simulink model "FullWave"  (R2024b)
settings: Solver=VariableStepAuto  StartTime=0.0  StopTime=s*(1/f)  RelTol=1e-9
model workspace (MAT data in the model file):
  E = 72
  L = 0.5
  R = 25
  Vll_rms = 480
  alpha = 30
  f = 60
  s = 1
libraries: spsMeanLib x18, eeRmsMeasurement x18, spsCurrentMeasurementLib x9, spsDiodeLib x9, spsThyristorLib x9, spsVoltageMeasurementLib x9, simulink x3, spsSeriesRLCBranchLib x3, spsThreePhaseSourceLib x3, sps_lib x1
settings Model: Creator=Mohammed Abdelrahman  LastModifiedBy=Mohammed Abdelrahman

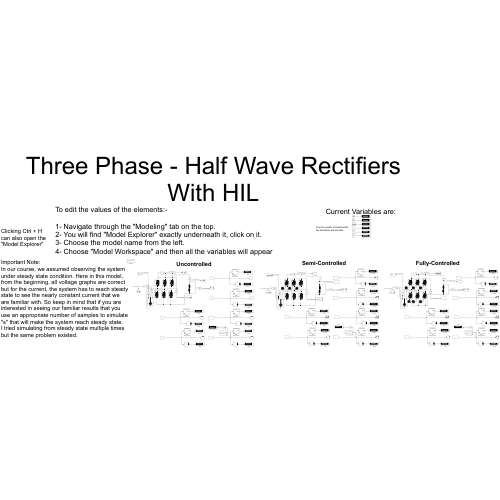
[thumbnail: Simulink's stored preview of the top-level diagram]
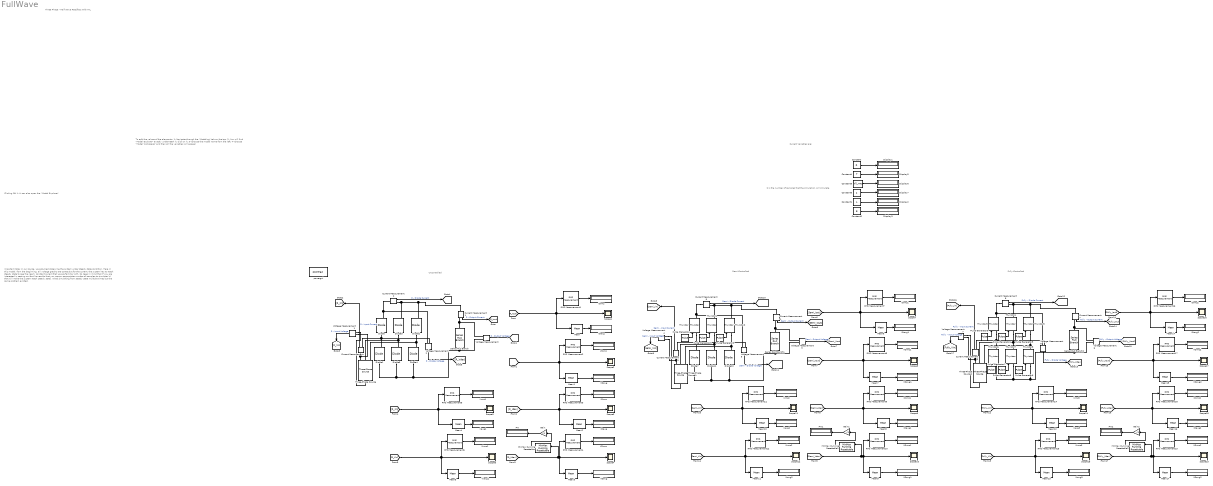
== system FullWave ==
  note: Important Note:
      | In our course, we assumed observing the system under steady state condition. Here in this model, from the beginning, all voltage graphs are correct but for the current, the system has to reach steady state to see the nearly constant current that we are familiar with. So keep in mind that if you are interested in seeing our familiar results that you use an appropriate number of samples to simulate "s" that will make the system reach steady state.
      | I tried simulating from steady state multiple times but the same problem existed.
  note: Clicking Ctrl + H can also open the "Model Explorer"
  note: S is the number of samples that the simulation will simulate
  note: Three Phase - Half Wave Rectifiers
      | With HIL
  note: To edit the values of the elements:-
      |
      | 1- Navigate through the "Modeling" tab on the top.
      | 2- You will find "Model Explorer" exactly underneath it, click on it.
      | 3- Choose the model name from the left.
      | 4- Choose "Model Workspace" and then all the variables will appear
  note: Uncontrolled
  note: Semi-Controlled
  note: Current Variables are:
  note: Fully-Controlled
  Constant : Constant  Value=R
  Constant1 : Constant  Value=L
  Constant2 : Constant  Value=E
  Constant4 : Constant  Value=f
  Constant5 : Constant  Value=Vll_rms
  Constant6 : Constant  Value=s
  Current Measurement{,1..8} (9 alike) : spsCurrentMeasurementLib/Current Measurement  PhasorSimulation=off  OutputType=Complex  PSBequivalent=0
  Diode{,1..5,7,10..11} (9 alike) : spsDiodeLib/Diode  Ron=0.001  Lon=0  Vf=0.0001  IC=0  UseSnubber=0  Rs=10e5  Cs=250e-9  Measurements=on
  Display{1..3,5..7} (6 alike) : Display
  Gain : Gain  Gain=-1
  Gain1 : Gain  Gain=-1
  Gain2 : Gain  Gain=-1
  IDavg : Display
  IDavg1 : Display
  IDavg2 : Display
  IDrms : Display
  IDrms1 : Display
  IDrms2 : Display
  IOavg : Display
  IOavg1 : Display
  IOavg2 : Display
  IOrms : Display
  IOrms1 : Display
  IOrms2 : Display
  Iiavg1 : Display
  Iiavg2 : Display
  Iiavg3 : Display
  Iirms1 : Display
  Iirms2 : Display
  Iirms3 : Display
  Mean{,1..17} (18 alike) : spsMeanLib/Mean  Freq=60  Vinit=0  Ts=0
  MinMax Running Resettable : simulink/Math Operations/MinMax Running Resettable  Function=min  vinit=0.0
  MinMax Running Resettable1 : simulink/Math Operations/MinMax Running Resettable  Function=min  vinit=0.0
  MinMax Running Resettable2 : simulink/Math Operations/MinMax Running Resettable  Function=min  vinit=0.0
  PIV : Display
  PIV1 : Display
  PIV2 : Display
  Pulse Generator : DiscretePulseGenerator  PulseType=Time based  Period=1/f  PulseWidth=5  PhaseDelay=(30+alpha)/(360*f)
  Pulse Generator1 : DiscretePulseGenerator  PulseType=Time based  Period=1/f  PulseWidth=5  PhaseDelay=(150+alpha)/(360*f)
  Pulse Generator2 : DiscretePulseGenerator  PulseType=Time based  Period=1/f  PulseWidth=5  PhaseDelay=(270+alpha)/(360*f)
  Pulse Generator3 : DiscretePulseGenerator  PulseType=Time based  Period=1/f  PulseWidth=5  PhaseDelay=(30+alpha)/(360*f)
  Pulse Generator4 : DiscretePulseGenerator  PulseType=Time based  Period=1/f  PulseWidth=5  PhaseDelay=(150+alpha)/(360*f)
  Pulse Generator5 : DiscretePulseGenerator  PulseType=Time based  Period=1/f  PulseWidth=5  PhaseDelay=(270+alpha)/(360*f)
  Pulse Generator6 : DiscretePulseGenerator  PulseType=Time based  Period=1/f  PulseWidth=5  PhaseDelay=(90+alpha)/(360*f)
  Pulse Generator7 : DiscretePulseGenerator  PulseType=Time based  Period=1/f  PulseWidth=5  PhaseDelay=(210+alpha)/(360*f)
  Pulse Generator8 : DiscretePulseGenerator  PulseType=Time based  Period=1/f  PulseWidth=5  PhaseDelay=(330+alpha)/(360*f)
  RMS Measurement{1..18} (18 alike) : eeRmsMeasurement/RMS Measurement  LabelModeActiveChoice=Total  F=f  SpecifyHarmonics=off  K=[0 1 2]  Ts=0
      settings: LibrarySourceBlock=|
      | ee_sl_lib/Measurements/RMS
      | Measurement
  Scope{1..18} (18 alike) : Scope
  Series RLC Branch : spsSeriesRLCBranchLib/Series RLC Branch  LConnTagsString=__new0  RConnTagsString=__new0  BranchType=RL  Resistance=R  Inductance=L  SetiL0=off  InitialCurrent=0  Capacitance=1e-6  Setx0=off  InitialVoltage=0  Measurements=None
  Series RLC Branch1 : spsSeriesRLCBranchLib/Series RLC Branch  LConnTagsString=__new0  RConnTagsString=__new0  BranchType=RL  Resistance=R  Inductance=L  SetiL0=off  InitialCurrent=0  Capacitance=1e-6  Setx0=off  InitialVoltage=0  Measurements=None
  Series RLC Branch2 : spsSeriesRLCBranchLib/Series RLC Branch  LConnTagsString=__new0  RConnTagsString=__new0  BranchType=RL  Resistance=R  Inductance=L  SetiL0=off  InitialCurrent=0  Capacitance=1e-6  Setx0=off  InitialVoltage=0  Measurements=None
  Three-Phase Source : spsThreePhaseSourceLib/Three-Phase Source  InternalConnection=Yn  VoltagePhases=off  Voltage=Vll_rms/sqrt(3)  PhaseAngle=0  Voltage_phases=[25e3 25e3 25e3]/sqrt(3)  PhaseAngles_phases=[0 -120 +120]  Frequency=f  NonIdealSource=off  SpecifyImpedance=off  Resistance=0.00001  Inductance=16.58e-6  ShortCircuitLevel=100e6  BaseVoltage=25e3  XRratio=7  BusType=swing  Pref=10e3  Qref=0  Prefabc=[10e3, 10e3, 10e3]  Qrefabc=[0, 0, 0]  Qmin=-inf  Qmax=inf
  Three-Phase Source1 : spsThreePhaseSourceLib/Three-Phase Source  InternalConnection=Yn  VoltagePhases=off  Voltage=Vll_rms/sqrt(3)  PhaseAngle=0  Voltage_phases=[25e3 25e3 25e3]/sqrt(3)  PhaseAngles_phases=[0 -120 +120]  Frequency=f  NonIdealSource=off  SpecifyImpedance=off  Resistance=0.00001  Inductance=16.58e-6  ShortCircuitLevel=100e6  BaseVoltage=25e3  XRratio=7  BusType=swing  Pref=10e3  Qref=0  Prefabc=[10e3, 10e3, 10e3]  Qrefabc=[0, 0, 0]  Qmin=-inf  Qmax=inf
  Three-Phase Source2 : spsThreePhaseSourceLib/Three-Phase Source  InternalConnection=Yn  VoltagePhases=off  Voltage=Vll_rms/sqrt(3)  PhaseAngle=0  Voltage_phases=[25e3 25e3 25e3]/sqrt(3)  PhaseAngles_phases=[0 -120 +120]  Frequency=f  NonIdealSource=off  SpecifyImpedance=off  Resistance=0.00001  Inductance=16.58e-6  ShortCircuitLevel=100e6  BaseVoltage=25e3  XRratio=7  BusType=swing  Pref=10e3  Qref=0  Prefabc=[10e3, 10e3, 10e3]  Qrefabc=[0, 0, 0]  Qmin=-inf  Qmax=inf
  Thyristor{,1..8} (9 alike) : spsThyristorLib/Thyristor  Ron=0.001  Lon=0  Vf=0.0001  IC=0  Rs=10e5  Cs=250e-9  Measurements=on
  VDavg : Display
  VDavg1 : Display
  VDavg2 : Display
  VDrms : Display
  VDrms1 : Display
  VDrms2 : Display
  VOavg : Display
  VOavg1 : Display
  VOavg2 : Display
  VOrms : Display
  VOrms1 : Display
  VOrms2 : Display
  Viavg1 : Display
  Viavg2 : Display
  Viavg3 : Display
  Virms1 : Display
  Virms2 : Display
  Virms3 : Display
  Voltage Measurement{,1..8} (9 alike) : spsVoltageMeasurementLib/Voltage Measurement  PhasorSimulation=off  OutputType=Complex  PSBequivalent=0
  powergui : sps_lib/powergui  Priority=1  SimulationMode=Continuous  SampleTime=50e-6  frequency=60  Iterations=50  frequencyindice=60  Pbase=100e6  ErrMax=1e-4  UnitsV=kV  UnitsW=MW  buscounter=0  FunctionMessages=off  echomessages=off  EnableUseOfTLC=off  CurrentSourceSwitches=off  DisableSnubberDevices=off  DisableRonSwitches=off  DisableVfSwitches=off  DisplayEquations=off  AutomaticDiscreteSolvers=off  SolverType=Tustin/Backward Euler (TBE)  Interpol=off  ExternalGateDelay=off  methode=off  Ts=100  x0status=steady  SPID=on  SwTol=0  HookPort=off  NonlinearTolerance=1e-4  nMaxIteration=100  ContinueOnMaxIteration=off  RestoreLinks=warning  ResistiveCurrentMeasurement=off  Frange=[0:2:500]  Ylog=off  Xlog=on  ShowGrid=off  save=off  variable=ZData  structure=0  ZoomFFT=off  StartTime=0.0  cycles=1  DisplayStyle=1  fundamental=60  FreqAxis=off  MaxFrequency=1000  frequencyindicesteady=1  RmsSteady=1  display=off
  wires:
  Current Measurement1/1 -> [R_Iout]  "R - Output Current"
  Voltage Measurement/1 -> [R_Vout]  "R - Output Voltage"
  Current Measurement/1 -> [R_Iin]  "R - Input Current"
  Voltage Measurement1/1 -> [R_Vin]  "R - Input Voltage"
  [R_Iout] -> Scope1/1, RMS Measurement1/1, Mean/1
  Mean1/1 -> VOavg/1
  Mean/1 -> IOavg/1
  [R_Vout] -> Mean1/1, RMS Measurement2/1, Scope2/1
  RMS Measurement2/1 -> VOrms/1
  RMS Measurement1/1 -> IOrms/1
  Voltage Measurement2/1 -> [R_Vdev]  "R - Diode Voltage"
  Current Measurement2/1 -> [R_Idev]  "R - Diode Current"
  [R_Vdev] -> RMS Measurement4/1, Scope4/1, Mean3/1, MinMax Running Resettable/1
  [R_Idev] -> Scope3/1, RMS Measurement3/1, Mean2/1
  RMS Measurement3/1 -> IDrms/1
  Mean3/1 -> VDavg/1
  Mean2/1 -> IDavg/1
  RMS Measurement4/1 -> VDrms/1
  Gain/1 -> PIV/1
  MinMax Running Resettable/1 -> Gain/1
  [R_Vin] -> Scope6/1, Mean5/1, RMS Measurement6/1
  [R_Iin] -> Scope5/1, RMS Measurement5/1, Mean4/1
  RMS Measurement5/1 -> Iirms1/1
  Mean5/1 -> Viavg1/1
  Mean4/1 -> Iiavg1/1
  RMS Measurement6/1 -> Virms1/1
  RMS Measurement12/1 -> Virms2/1
  [Semi_Vout] -> Mean7/1, RMS Measurement8/1, Scope8/1
  [Semi_Iout] -> Scope7/1, RMS Measurement7/1, Mean6/1
  RMS Measurement9/1 -> IDrms1/1
  RMS Measurement10/1 -> VDrms1/1
  [Semi_Idev] -> Scope9/1, RMS Measurement9/1, Mean8/1
  Gain1/1 -> PIV1/1
  Mean9/1 -> VDavg1/1
  [Semi_Vin] -> Mean11/1, RMS Measurement12/1, Scope12/1
  [Semi_Vdev] -> RMS Measurement10/1, Scope10/1, Mean9/1, MinMax Running Resettable1/1
  RMS Measurement8/1 -> VOrms1/1
  MinMax Running Resettable1/1 -> Gain1/1
  Mean6/1 -> IOavg1/1
  Mean7/1 -> VOavg1/1
  RMS Measurement7/1 -> IOrms1/1
  RMS Measurement11/1 -> Iirms2/1
  Mean10/1 -> Iiavg2/1
  Mean11/1 -> Viavg2/1
  Mean8/1 -> IDavg1/1
  [Semi_Iin] -> Scope11/1, RMS Measurement11/1, Mean10/1
  Constant5/1 -> Display6/1
  Constant/1 -> Display1/1
  Constant6/1 -> Display7/1
  Constant1/1 -> Display2/1
  Constant4/1 -> Display5/1
  Constant2/1 -> Display3/1
  Voltage Measurement4/1 -> [Semi_Vin]  "Semi - Input Voltage"
  Voltage Measurement3/1 -> [Semi_Vout]  "Semi - Output Voltage"
  Current Measurement5/1 -> [Semi_Idev]  "Semi - Diode Current"
  Voltage Measurement5/1 -> [Semi_Vdev]  "Semi - Diode Voltage"
  Current Measurement3/1 -> [Semi_Iin]  "Semi - Input Current"
  Current Measurement4/1 -> [Semi_Iout]  "Semi - Output Current"
  Pulse Generator/1 -> Thyristor/1
  Pulse Generator1/1 -> Thyristor1/1
  Pulse Generator2/1 -> Thyristor2/1
  Mean12/1 -> Iiavg3/1
  RMS Measurement13/1 -> VDrms2/1
  RMS Measurement14/1 -> Iirms3/1
  [Fully_Idev] -> Scope18/1, RMS Measurement18/1, Mean16/1
  MinMax Running Resettable2/1 -> Gain2/1
  Mean14/1 -> IOavg2/1
  Gain2/1 -> PIV2/1
  [Fully_Vdev] -> RMS Measurement13/1, Scope13/1, Mean17/1, MinMax Running Resettable2/1
  [Fully_Iin] -> Scope14/1, RMS Measurement14/1, Mean12/1
  Mean16/1 -> IDavg2/1
  [Fully_Vin] -> Mean13/1, RMS Measurement15/1, Scope15/1
  RMS Measurement15/1 -> Virms3/1
  [Fully_Iout] -> Scope16/1, RMS Measurement16/1, Mean14/1
  Mean13/1 -> Viavg3/1
  Mean17/1 -> VDavg2/1
  [Fully_Vout] -> Mean15/1, RMS Measurement17/1, Scope17/1
  Mean15/1 -> VOavg2/1
  RMS Measurement18/1 -> IDrms2/1
  RMS Measurement16/1 -> IOrms2/1
  RMS Measurement17/1 -> VOrms2/1
  Pulse Generator4/1 -> Thyristor4/1
  Current Measurement6/1 -> [Fully_Iin]  "Fully - Input Current"
  Voltage Measurement7/1 -> [Fully_Vin]  "Fully - Input Voltage"
  Current Measurement8/1 -> [Fully_Idev]  "Fully - Diode Current"
  Voltage Measurement6/1 -> [Fully_Vout]  "Fully - Output Voltage"
  Pulse Generator3/1 -> Thyristor3/1
  Current Measurement7/1 -> [Fully_Iout]  "Fully - Output Current"
  Voltage Measurement8/1 -> [Fully_Vdev]  "Fully - Diode Voltage"
  Pulse Generator5/1 -> Thyristor5/1
  Pulse Generator6/1 -> Thyristor8/1
  Pulse Generator7/1 -> Thyristor6/1
  Pulse Generator8/1 -> Thyristor7/1
  connections:
  Series RLC Branch/LConn1 -- Voltage Measurement/LConn1 -- Current Measurement1/RConn1
  Current Measurement2/RConn1 -- Diode2/RConn1 -- Current Measurement1/LConn1 -- Diode3/RConn1
  Voltage Measurement2/LConn1 -- Current Measurement/RConn1 -- Diode1/RConn1 -- Diode/LConn1
  Diode/RConn1 -- Voltage Measurement2/LConn2 -- Current Measurement2/LConn1
  Current Measurement/LConn1 -- Voltage Measurement1/LConn1 -- Three-Phase Source/RConn1
  Voltage Measurement/LConn2 -- Diode1/LConn1 -- Diode5/LConn1 -- Diode4/LConn1 -- Series RLC Branch/RConn1
  Diode3/LConn1 -- Three-Phase Source/RConn2 -- Diode5/RConn1
  Diode2/LConn1 -- Three-Phase Source/RConn3 -- Diode4/RConn1
  Voltage Measurement1/LConn2 -- Three-Phase Source/LConn1
  Current Measurement5/LConn1 -- Voltage Measurement5/LConn2 -- Thyristor/RConn1
  Diode11/LConn1 -- Diode7/LConn1 -- Diode10/LConn1 -- Voltage Measurement3/LConn2 -- Series RLC Branch1/RConn1
  Voltage Measurement5/LConn1 -- Thyristor/LConn1 -- Current Measurement3/RConn1 -- Diode7/RConn1
  Current Measurement5/RConn1 -- Current Measurement4/LConn1 -- Thyristor2/RConn1 -- Thyristor1/RConn1
  Diode11/RConn1 -- Thyristor1/LConn1 -- Three-Phase Source1/RConn2
  Current Measurement3/LConn1 -- Voltage Measurement4/LConn1 -- Three-Phase Source1/RConn1
  Diode10/RConn1 -- Thyristor2/LConn1 -- Three-Phase Source1/RConn3
  Voltage Measurement3/LConn1 -- Current Measurement4/RConn1 -- Series RLC Branch1/LConn1
  Voltage Measurement4/LConn2 -- Three-Phase Source1/LConn1
  Voltage Measurement6/LConn1 -- Current Measurement7/RConn1 -- Series RLC Branch2/LConn1
  Three-Phase Source2/RConn3 -- Thyristor5/LConn1 -- Thyristor8/RConn1
  Three-Phase Source2/RConn2 -- Thyristor7/RConn1 -- Thyristor4/LConn1
  Series RLC Branch2/RConn1 -- Thyristor7/LConn1 -- Thyristor6/LConn1 -- Thyristor8/LConn1 -- Voltage Measurement6/LConn2
  Thyristor5/RConn1 -- Current Measurement8/RConn1 -- Thyristor4/RConn1 -- Current Measurement7/LConn1
  Voltage Measurement8/LConn1 -- Thyristor6/RConn1 -- Thyristor3/LConn1 -- Current Measurement6/RConn1
  Current Measurement6/LConn1 -- Voltage Measurement7/LConn1 -- Three-Phase Source2/RConn1
  Current Measurement8/LConn1 -- Voltage Measurement8/LConn2 -- Thyristor3/RConn1
  Voltage Measurement7/LConn2 -- Three-Phase Source2/LConn1
